simulink model "Chapter6_Discret_AP"  (R2024b)
settings: Solver=ode4  StartTime=0.0  StopTime=SIM.StopTime  FixedStep=SIM.FixedStepSize  RelTol=1e-3
values from neighbouring files (symbols this model uses):
  AP = computeAutopilotGains(MAV, TRIM, TFS, DES)    [ch6_main.m]    (also in computeAutopilotGains.m = struct())
  CMD = struct()    [ch6_main.m]
  DES = loadDesignParams()    [ch6_main.m]    (also in loadDesignParams.m = struct())
  LIM = loadSafetyLimits()    [ch6_main.m]
  TRIM =     [ch6.mat]    (also in ch6_main.m = findTrim(TRIM_MODEL, Va_trim, R_trim, gamma_trim, TRIM_DATA_; findTrim.m = struct())
  WIND = loadWindParameters()    [ch6_main.m]
undefined symbols (not defined in the file or in its folder): DiscIntNeverNeededParam, drawAircraft, F, Light, MAV, MIL, plotter, SIM
libraries: simulink x11, matrix_library x2, aerolibwind2 x1
(part 2 of 2)

== matlab function Chapter6_Discret_AP/Autopilot/Longitudinal Autopilot/MATLAB Function ==
  data: h_cmd input; zone output; h input; DES parameter
function zone = determineZone(h_cmd, h, DES)
    persistent current_zone;
    
    % --- SMART INITIALIZATION ---
    if isempty(current_zone)
        if h < DES.Altitude.Takeoff 
            current_zone = 0; % Take-off
        else
            current_zone = 2; % Hold
        end
    end
    
    err = h_cmd - h;
    enter_threshold = DES.Altitude.Threshold; 
    exit_threshold  = enter_threshold / 2; % Hysteresis
    
    % --- STATE MACHINE ---
    switch current_zone
        
        case 0 % --- TAKE-OFF ZONE ---
            if h > DES.Altitude.Takeoff
                current_zone = 1; % Climb Zone'a geç
            end

        case 1 % --- CLIMB ZONE ---
            if err < exit_threshold
                current_zone = 2; 
            end
            
        case 2 % --- HOLD ZONE --- 
            if err > enter_threshold
                current_zone = 1; % Climb
            elseif err < -enter_threshold
                current_zone = 3; % Descend
            end
            
        case 3 % --- DESCEND ZONE ---
            if err > -exit_threshold
                current_zone = 2; % Hold'a geç
            end
            
        otherwise
            current_zone = 2;
    end
    
    zone = current_zone;
end

== matlab function Chapter6_Discret_AP/Plant/Atmospheric Effects/Aerodynamic Effect on Longitudinal Motion/Variant Subsystem/Nonlinear Lift Drag Effect of Alpha/Equation 4.10 ==
  data: alpha input; lambda1 output; MAV parameter; lambda2 output
function [lambda1, lambda2] = fcn(alpha, MAV)
% Equation 4.9 - 4.10    
exp_m = exp(-MAV.M * (alpha - MAV.alpha_0));
exp_p = exp(MAV.M * (alpha + MAV.alpha_0));
lambda2 = ( 1 + exp_m + exp_p) / ((1 + exp_m)*(1 + exp_p));
lambda1 = 1 - lambda2;
end

== matlab function Chapter6_Discret_AP/Plant/Gravitational Force/R_B_I_c3 ==
  data: u input; y output
function y = fcn(u)
    y = zeros(3,1);
    y(1) = -sin(u(2));
    y(2) = cos(u(2)) * sin(u(1));
    y(3) = cos(u(2)) * cos(u(1));
end

== matlab function Chapter6_Discret_AP/Plant/Subsystem1/MATLAB Function ==
  data: u input; y output
function y = fcn(u)
    y = wrapToPi(u);

== matlab function Chapter6_Discret_AP/Plant/Subsystem1/Subsystem/MATLAB Function ==
  data: u input; y output
function y = fcn(u)
    sphi = sin(u(1));
    cphi = cos(u(1));

    sthe = sin(u(2));
    cthe = cos(u(2));

    scthe = 1 / cthe;
    tthe = scthe * sthe;

    y = [1 sphi * tthe cphi*tthe;
         0 cphi -sphi;
         0 sphi*scthe cphi*scthe];

== matlab function Chapter6_Discret_AP/Autopilot/Lateral Autopilot/Sideslip Hold Control Loop/MATLAB Function ==
  data: u_unsat input; I output; u_sat input; Ki_e input
function I = clampAntiWindup(u_unsat, u_sat, Ki_e)
    is_saturated = (u_unsat ~= u_sat);
    is_same_dir = (u_unsat * Ki_e > 0);

    if (is_saturated && is_same_dir), I = 0;
    else, I = Ki_e;
    end
end

== matlab function Chapter6_Discret_AP/Autopilot/Lateral Autopilot/Course Hold Control Loop/MATLAB Function ==
  data: u_unsat input; I output; u_sat input; Ki_e input
function I = clampAntiWindup(u_unsat, u_sat, Ki_e)
    is_saturated = (u_unsat ~= u_sat);
    is_same_dir = (u_unsat * Ki_e > 0);

    if (is_saturated && is_same_dir), I = 0;
    else, I = Ki_e;
    end
end

== matlab function Chapter6_Discret_AP/Autopilot/Lateral Autopilot/Course Hold Control Loop/Roll Hold Control Loop/MATLAB Function ==
  data: u_unsat input; I output; u_sat input; Ki_e input
function I = clampAntiWindup(u_unsat, u_sat, Ki_e)
    is_saturated = (u_unsat ~= u_sat);
    is_same_dir = (u_unsat * Ki_e > 0);

    if (is_saturated && is_same_dir), I = 0;
    else, I = Ki_e;
    end
end

== matlab function Chapter6_Discret_AP/Autopilot/Longitudinal Autopilot/Altitude Hold Control Outer Loop/MATLAB Function ==
  data: u_unsat input; I output; u_sat input; Ki_e input
function I = clampAntiWindup(u_unsat, u_sat, Ki_e)
    is_saturated = (u_unsat ~= u_sat);
    is_same_dir = (u_unsat * Ki_e > 0);

    if (is_saturated && is_same_dir), I = 0;
    else, I = Ki_e;
    end
end

== matlab function Chapter6_Discret_AP/Autopilot/Longitudinal Autopilot/Airspeed Hold Control using Pitch Outer Loop/MATLAB Function ==
  data: u_unsat input; I output; u_sat input; Ki_e input
function I = clampAntiWindup(u_unsat, u_sat, Ki_e)
    is_saturated = (u_unsat ~= u_sat);
    is_same_dir = (u_unsat * Ki_e > 0);

    if (is_saturated && is_same_dir), I = 0;
    else, I = Ki_e;
    end
end

== matlab function Chapter6_Discret_AP/Autopilot/Longitudinal Autopilot/Airspeed Hold Control using Throttle /MATLAB Function ==
  data: u_unsat input; I output; u_sat input; Ki_e input
function I = clampAntiWindup(u_unsat, u_sat, Ki_e)
    is_saturated = (u_unsat ~= u_sat);
    is_same_dir = (u_unsat * Ki_e > 0);

    if (is_saturated && is_same_dir), I = 0;
    else, I = Ki_e;
    end
end
